simulink model "BCfirsttestwithLPfilter_Simulation"  (Simulink 6.4)
settings: Solver=FixedStepDiscrete  StartTime=0.0  StopTime=1  FixedStep=1/300  RelTol=1e-3
libraries: dspsigops x50
settings Model: Creator=Casparus  LastModifiedBy=lubink
settings OptimizationCC: InlineParams=on  InlineInvariantSignals=on  EnforceIntegerDowncast=off  ZeroExternalMemoryAtStartup=off  ZeroInternalMemoryAtStartup=off  InitFltsAndDblsToZero=off  EfficientFloat2IntCast=on  OptimizeModelRefInitCode=on  LifeSpan=1
settings DebuggingCC: SignalInfNanChecking=error  ReadBeforeWriteMsg=EnableAllAsError  WriteAfterWriteMsg=EnableAllAsError  WriteAfterReadMsg=EnableAllAsError  AlgebraicLoopMsg=error  ArtificialAlgebraicLoopMsg=error  CheckExecutionContextPreStartOutputMsg=on  CheckExecutionContextRuntimeOutputMsg=on  SignalResolutionControl=UseLocalSettings  BlockPriorityViolationMsg=error  SolverPrmCheckMsg=error  InheritedTsInSrcMsg=error  DiscreteInheritContinuousMsg=error  MultiTaskDSMMsg=error  MultiTaskCondExecSysMsg=error  SigSpecEnsureSampleTimeMsg=error  CheckMatrixSingularityMsg=error  ParameterUnderflowMsg=error  ParameterPrecisionLossMsg=error  UnderSpecifiedDataTypeMsg=error  UnnecessaryDatatypeConvMsg=warning  VectorMatrixConversionMsg=error  FcnCallInpInsideContextMsg=Enable All  SignalLabelMismatchMsg=error  UnconnectedInputMsg=error  UnconnectedOutputMsg=error  UnconnectedLineMsg=error  SFcnCompatibilityMsg=error  BusObjectLabelMismatch=error  RootOutportRequireBusObject=error  AssertControl=DisableAll  ModelReferenceIOMsg=error  ModelReferenceIOMismatchMessage=error  ModelReferenceCSMismatchMessage=warning  UnknownTsInhSupMsg=error  ModelReferenceDataLoggingMessage=error
settings HardwareCC: ProdBitPerInt=16  ProdEndianess=LittleEndian  ProdWordSize=16  ProdHWDeviceType=16-bit Generic  TargetHWDeviceType=32-bit Generic
settings RTWCC: SystemTargetFile=dspic.tlc  TemplateMakefile=dspic_pic30_gcc.tmf  PostCodeGenCommand=dsPIC_Compile()  Description=Embedded Target for Microchip dsPIC (real-time)  ProcessScript=dspic_make_rtw_hook
settings CodeAppCC: ForceParamTrailComments=on  IgnoreCustomStorageClasses=off  MangleLength=4  ReqsInCode=on
settings STFCustomTargetCC: TargetFcnLib=ansi_tfl_tmw.mat  GenFloatMathFcnCalls=ANSI_C  ModelReferenceCompliant=off  IncludeMdlTerminateFcn=off  CombineOutputUpdateFcns=on  SuppressErrorStatus=on  ERTCustomFileBanners=on  SupportContinuousTime=off  SupportNonInlinedSFcns=off  SystemTargetFile=dspic.tlc
settings ERTTargetCC: TargetFcnLib=ansi_tfl_tmw.mat  GenFloatMathFcnCalls=ANSI_C  ModelReferenceCompliant=off  CompOptLevelCompliant=off  IncludeMdlTerminateFcn=off  SuppressErrorStatus=on  ModelStepFunctionPrototypeControlCompliant=off  ExtModeMexFile=ext_serial_win32_comm  InlinedParameterPlacement=NonHierarchical  ERTSrcFileBannerTemplate=dsPIC_code_template.cgt  ERTHdrFileBannerTemplate=dsPIC_code_template.cgt  ERTDataSrcFileTemplate=dsPIC_code_template.cgt  ERTDataHdrFileTemplate=dsPIC_code_template.cgt  ERTCustomFileTemplate=dsPIC_main.tlc
settings CustomProperty: DataType=string  Value=C:\PROGRA~1\MATLAB\R2007b\bin\win32\gmake

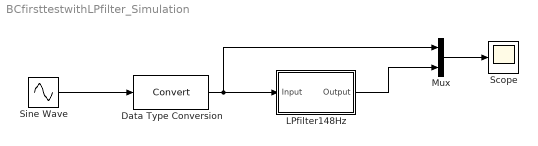
== system BCfirsttestwithLPfilter_Simulation ==
  Data Type Conversion : DataTypeConversion  OutDataTypeMode=uint8  SaturateOnIntegerOverflow=on
  LPfilter148Hz : Subsystem  Tag=FilterWizardSubSystem
      settings: ErrorFcn=dspFilterRealizedInBasicElemsAlgLoopErrFcnCallback
  Mux : Mux  Inputs=2
  Scope : Scope
  Sine Wave : Sin  Amplitude=50  Bias=100  Frequency=30*2*pi  SampleTime=1/300
  wires:
  Sine Wave/1 -> Data Type Conversion/1
  Data Type Conversion/1 -> LPfilter148Hz/1(Input), Mux/1
  LPfilter148Hz/1(Output) -> Mux/2
  Mux/1 -> Scope/1

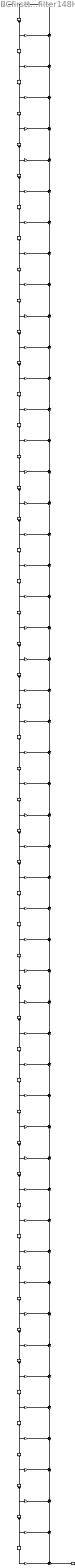
== system BCfirsttestwithLPfilter_Simulation/LPfilter148Hz ==
  Input : Inport
  BodyDelay{2..51} (50 alike) : dspsigops/Delay  Orientation=down  dly_unit=Samples  delay=1  ic_detail=off  dif_ic_for_ch=off  dif_ic_for_dly=off  ic=0  reset_popup=None
  BodyLSum{2..50} (49 alike) : Sum  Orientation=down  Inputs=++|  OutScaling=1  RndMeth=Nearest  SaturateOnIntegerOverflow=on
  BodyLSum51 : Sum  Inputs=++|  OutScaling=1  RndMeth=Nearest  SaturateOnIntegerOverflow=on
  b(1) : Gain  Gain=0.014552788094050004  ParameterDataTypeMode=Specify via dialog  ParameterDataType=float('double')  OutScaling=1  RndMeth=Nearest  SaturateOnIntegerOverflow=on
  b(10) : Gain  Gain=0.009640191238745691  ParameterDataTypeMode=Specify via dialog  ParameterDataType=float('double')  OutScaling=1  RndMeth=Nearest  SaturateOnIntegerOverflow=on
  b(11) : Gain  Gain=-0.0085605708557222188  ParameterDataTypeMode=Specify via dialog  ParameterDataType=float('double')  OutScaling=1  RndMeth=Nearest  SaturateOnIntegerOverflow=on
  b(12) : Gain  Gain=0.0063507327962420345  ParameterDataTypeMode=Specify via dialog  ParameterDataType=float('double')  OutScaling=1  RndMeth=Nearest  SaturateOnIntegerOverflow=on
  b(13) : Gain  Gain=-0.0029026251186017836  ParameterDataTypeMode=Specify via dialog  ParameterDataType=float('double')  OutScaling=1  RndMeth=Nearest  SaturateOnIntegerOverflow=on
  b(14) : Gain  Gain=-0.0018214634792136299  ParameterDataTypeMode=Specify via dialog  ParameterDataType=float('double')  OutScaling=1  RndMeth=Nearest  SaturateOnIntegerOverflow=on
  b(15) : Gain  Gain=0.0077807436385992461  ParameterDataTypeMode=Specify via dialog  ParameterDataType=float('double')  OutScaling=1  RndMeth=Nearest  SaturateOnIntegerOverflow=on
  b(16) : Gain  Gain=-0.014854401199296334  ParameterDataTypeMode=Specify via dialog  ParameterDataType=float('double')  OutScaling=1  RndMeth=Nearest  SaturateOnIntegerOverflow=on
  b(17) : Gain  Gain=0.022857994519878629  ParameterDataTypeMode=Specify via dialog  ParameterDataType=float('double')  OutScaling=1  RndMeth=Nearest  SaturateOnIntegerOverflow=on
  b(18) : Gain  Gain=-0.031505854072013589  ParameterDataTypeMode=Specify via dialog  ParameterDataType=float('double')  OutScaling=1  RndMeth=Nearest  SaturateOnIntegerOverflow=on
  b(19) : Gain  Gain=0.040407776537517141  ParameterDataTypeMode=Specify via dialog  ParameterDataType=float('double')  OutScaling=1  RndMeth=Nearest  SaturateOnIntegerOverflow=on
  b(2) : Gain  Gain=0.001488942337451464  ParameterDataTypeMode=Specify via dialog  ParameterDataType=float('double')  OutScaling=1  RndMeth=Nearest  SaturateOnIntegerOverflow=on
  b(20) : Gain  Gain=-0.049274632193230417  ParameterDataTypeMode=Specify via dialog  ParameterDataType=float('double')  OutScaling=1  RndMeth=Nearest  SaturateOnIntegerOverflow=on
  b(21) : Gain  Gain=0.057661319766925831  ParameterDataTypeMode=Specify via dialog  ParameterDataType=float('double')  OutScaling=1  RndMeth=Nearest  SaturateOnIntegerOverflow=on
  b(22) : Gain  Gain=-0.065171220365631818  ParameterDataTypeMode=Specify via dialog  ParameterDataType=float('double')  OutScaling=1  RndMeth=Nearest  SaturateOnIntegerOverflow=on
  b(23) : Gain  Gain=0.0714398868910541  ParameterDataTypeMode=Specify via dialog  ParameterDataType=float('double')  OutScaling=1  RndMeth=Nearest  SaturateOnIntegerOverflow=on
  b(24) : Gain  Gain=-0.076157677489708669  ParameterDataTypeMode=Specify via dialog  ParameterDataType=float('double')  OutScaling=1  RndMeth=Nearest  SaturateOnIntegerOverflow=on
  b(25) : Gain  Gain=0.079087854814890529  ParameterDataTypeMode=Specify via dialog  ParameterDataType=float('double')  OutScaling=1  RndMeth=Nearest  SaturateOnIntegerOverflow=on
  b(26) : Gain  Gain=0.91991847348550915  ParameterDataTypeMode=Specify via dialog  ParameterDataType=float('double')  OutScaling=1  RndMeth=Nearest  SaturateOnIntegerOverflow=on
  b(27) : Gain  Gain=0.079087854814890529  ParameterDataTypeMode=Specify via dialog  ParameterDataType=float('double')  OutScaling=1  RndMeth=Nearest  SaturateOnIntegerOverflow=on
  b(28) : Gain  Gain=-0.076157677489708669  ParameterDataTypeMode=Specify via dialog  ParameterDataType=float('double')  OutScaling=1  RndMeth=Nearest  SaturateOnIntegerOverflow=on
  b(29) : Gain  Gain=0.0714398868910541  ParameterDataTypeMode=Specify via dialog  ParameterDataType=float('double')  OutScaling=1  RndMeth=Nearest  SaturateOnIntegerOverflow=on
  b(3) : Gain  Gain=-0.0022367192816874449  ParameterDataTypeMode=Specify via dialog  ParameterDataType=float('double')  OutScaling=1  RndMeth=Nearest  SaturateOnIntegerOverflow=on
  b(30) : Gain  Gain=-0.065171220365631818  ParameterDataTypeMode=Specify via dialog  ParameterDataType=float('double')  OutScaling=1  RndMeth=Nearest  SaturateOnIntegerOverflow=on
  b(31) : Gain  Gain=0.057661319766925831  ParameterDataTypeMode=Specify via dialog  ParameterDataType=float('double')  OutScaling=1  RndMeth=Nearest  SaturateOnIntegerOverflow=on
  b(32) : Gain  Gain=-0.049274632193230417  ParameterDataTypeMode=Specify via dialog  ParameterDataType=float('double')  OutScaling=1  RndMeth=Nearest  SaturateOnIntegerOverflow=on
  b(33) : Gain  Gain=0.040407776537517141  ParameterDataTypeMode=Specify via dialog  ParameterDataType=float('double')  OutScaling=1  RndMeth=Nearest  SaturateOnIntegerOverflow=on
  b(34) : Gain  Gain=-0.031505854072013589  ParameterDataTypeMode=Specify via dialog  ParameterDataType=float('double')  OutScaling=1  RndMeth=Nearest  SaturateOnIntegerOverflow=on
  b(35) : Gain  Gain=0.022857994519878629  ParameterDataTypeMode=Specify via dialog  ParameterDataType=float('double')  OutScaling=1  RndMeth=Nearest  SaturateOnIntegerOverflow=on
  b(36) : Gain  Gain=-0.014854401199296334  ParameterDataTypeMode=Specify via dialog  ParameterDataType=float('double')  OutScaling=1  RndMeth=Nearest  SaturateOnIntegerOverflow=on
  b(37) : Gain  Gain=0.0077807436385992461  ParameterDataTypeMode=Specify via dialog  ParameterDataType=float('double')  OutScaling=1  RndMeth=Nearest  SaturateOnIntegerOverflow=on
  b(38) : Gain  Gain=-0.0018214634792136299  ParameterDataTypeMode=Specify via dialog  ParameterDataType=float('double')  OutScaling=1  RndMeth=Nearest  SaturateOnIntegerOverflow=on
  b(39) : Gain  Gain=-0.0029026251186017836  ParameterDataTypeMode=Specify via dialog  ParameterDataType=float('double')  OutScaling=1  RndMeth=Nearest  SaturateOnIntegerOverflow=on
  b(4) : Gain  Gain=0.0033999777744855996  ParameterDataTypeMode=Specify via dialog  ParameterDataType=float('double')  OutScaling=1  RndMeth=Nearest  SaturateOnIntegerOverflow=on
  b(40) : Gain  Gain=0.0063507327962420345  ParameterDataTypeMode=Specify via dialog  ParameterDataType=float('double')  OutScaling=1  RndMeth=Nearest  SaturateOnIntegerOverflow=on
  b(41) : Gain  Gain=-0.0085605708557222188  ParameterDataTypeMode=Specify via dialog  ParameterDataType=float('double')  OutScaling=1  RndMeth=Nearest  SaturateOnIntegerOverflow=on
  b(42) : Gain  Gain=0.009640191238745691  ParameterDataTypeMode=Specify via dialog  ParameterDataType=float('double')  OutScaling=1  RndMeth=Nearest  SaturateOnIntegerOverflow=on
  b(43) : Gain  Gain=-0.0097539264573168211  ParameterDataTypeMode=Specify via dialog  ParameterDataType=float('double')  OutScaling=1  RndMeth=Nearest  SaturateOnIntegerOverflow=on
  b(44) : Gain  Gain=0.0091052834705578258  ParameterDataTypeMode=Specify via dialog  ParameterDataType=float('double')  OutScaling=1  RndMeth=Nearest  SaturateOnIntegerOverflow=on
  b(45) : Gain  Gain=-0.0079195888626813621  ParameterDataTypeMode=Specify via dialog  ParameterDataType=float('double')  OutScaling=1  RndMeth=Nearest  SaturateOnIntegerOverflow=on
  b(46) : Gain  Gain=0.0064281050997838478  ParameterDataTypeMode=Specify via dialog  ParameterDataType=float('double')  OutScaling=1  RndMeth=Nearest  SaturateOnIntegerOverflow=on
  b(47) : Gain  Gain=-0.0048540570262981418  ParameterDataTypeMode=Specify via dialog  ParameterDataType=float('double')  OutScaling=1  RndMeth=Nearest  SaturateOnIntegerOverflow=on
  b(48) : Gain  Gain=0.0033999777744855996  ParameterDataTypeMode=Specify via dialog  ParameterDataType=float('double')  OutScaling=1  RndMeth=Nearest  SaturateOnIntegerOverflow=on
  b(49) : Gain  Gain=-0.0022367192816874449  ParameterDataTypeMode=Specify via dialog  ParameterDataType=float('double')  OutScaling=1  RndMeth=Nearest  SaturateOnIntegerOverflow=on
  b(5) : Gain  Gain=-0.0048540570262981418  ParameterDataTypeMode=Specify via dialog  ParameterDataType=float('double')  OutScaling=1  RndMeth=Nearest  SaturateOnIntegerOverflow=on
  b(50) : Gain  Gain=0.001488942337451464  ParameterDataTypeMode=Specify via dialog  ParameterDataType=float('double')  OutScaling=1  RndMeth=Nearest  SaturateOnIntegerOverflow=on
  b(51) : Gain  Gain=0.014552788094050004  ParameterDataTypeMode=Specify via dialog  ParameterDataType=float('double')  OutScaling=1  RndMeth=Nearest  SaturateOnIntegerOverflow=on
  b(6) : Gain  Gain=0.0064281050997838478  ParameterDataTypeMode=Specify via dialog  ParameterDataType=float('double')  OutScaling=1  RndMeth=Nearest  SaturateOnIntegerOverflow=on
  b(7) : Gain  Gain=-0.0079195888626813621  ParameterDataTypeMode=Specify via dialog  ParameterDataType=float('double')  OutScaling=1  RndMeth=Nearest  SaturateOnIntegerOverflow=on
  b(8) : Gain  Gain=0.0091052834705578258  ParameterDataTypeMode=Specify via dialog  ParameterDataType=float('double')  OutScaling=1  RndMeth=Nearest  SaturateOnIntegerOverflow=on
  b(9) : Gain  Gain=-0.0097539264573168211  ParameterDataTypeMode=Specify via dialog  ParameterDataType=float('double')  OutScaling=1  RndMeth=Nearest  SaturateOnIntegerOverflow=on
  Output : Outport
  wires:
  BodyLSum51/1 -> Output/1
  b(51)/1 -> BodyLSum51/2
  BodyDelay51/1 -> b(51)/1
  BodyLSum50/1 -> BodyLSum51/1
  b(50)/1 -> BodyLSum50/1
  BodyDelay50/1 -> BodyDelay51/1, b(50)/1
  BodyLSum49/1 -> BodyLSum50/2
  b(49)/1 -> BodyLSum49/1
  BodyDelay49/1 -> BodyDelay50/1, b(49)/1
  BodyLSum48/1 -> BodyLSum49/2
  b(48)/1 -> BodyLSum48/1
  BodyDelay48/1 -> BodyDelay49/1, b(48)/1
  BodyLSum47/1 -> BodyLSum48/2
  b(47)/1 -> BodyLSum47/1
  BodyDelay47/1 -> BodyDelay48/1, b(47)/1
  BodyLSum46/1 -> BodyLSum47/2
  b(46)/1 -> BodyLSum46/1
  BodyDelay46/1 -> BodyDelay47/1, b(46)/1
  BodyLSum45/1 -> BodyLSum46/2
  b(45)/1 -> BodyLSum45/1
  BodyDelay45/1 -> BodyDelay46/1, b(45)/1
  BodyLSum44/1 -> BodyLSum45/2
  b(44)/1 -> BodyLSum44/1
  BodyDelay44/1 -> BodyDelay45/1, b(44)/1
  BodyLSum43/1 -> BodyLSum44/2
  b(43)/1 -> BodyLSum43/1
  BodyDelay43/1 -> BodyDelay44/1, b(43)/1
  BodyLSum42/1 -> BodyLSum43/2
  b(42)/1 -> BodyLSum42/1
  BodyDelay42/1 -> BodyDelay43/1, b(42)/1
  BodyLSum41/1 -> BodyLSum42/2
  b(41)/1 -> BodyLSum41/1
  BodyDelay41/1 -> BodyDelay42/1, b(41)/1
  BodyLSum40/1 -> BodyLSum41/2
  b(40)/1 -> BodyLSum40/1
  BodyDelay40/1 -> BodyDelay41/1, b(40)/1
  BodyLSum39/1 -> BodyLSum40/2
  b(39)/1 -> BodyLSum39/1
  BodyDelay39/1 -> BodyDelay40/1, b(39)/1
  BodyLSum38/1 -> BodyLSum39/2
  b(38)/1 -> BodyLSum38/1
  BodyDelay38/1 -> BodyDelay39/1, b(38)/1
  BodyLSum37/1 -> BodyLSum38/2
  b(37)/1 -> BodyLSum37/1
  BodyDelay37/1 -> BodyDelay38/1, b(37)/1
  BodyLSum36/1 -> BodyLSum37/2
  b(36)/1 -> BodyLSum36/1
  BodyDelay36/1 -> BodyDelay37/1, b(36)/1
  BodyLSum35/1 -> BodyLSum36/2
  b(35)/1 -> BodyLSum35/1
  BodyDelay35/1 -> BodyDelay36/1, b(35)/1
  BodyLSum34/1 -> BodyLSum35/2
  b(34)/1 -> BodyLSum34/1
  BodyDelay34/1 -> BodyDelay35/1, b(34)/1
  BodyLSum33/1 -> BodyLSum34/2
  b(33)/1 -> BodyLSum33/1
  BodyDelay33/1 -> BodyDelay34/1, b(33)/1
  BodyLSum32/1 -> BodyLSum33/2
  b(32)/1 -> BodyLSum32/1
  BodyDelay32/1 -> BodyDelay33/1, b(32)/1
  BodyLSum31/1 -> BodyLSum32/2
  b(31)/1 -> BodyLSum31/1
  BodyDelay31/1 -> BodyDelay32/1, b(31)/1
  BodyLSum30/1 -> BodyLSum31/2
  b(30)/1 -> BodyLSum30/1
  BodyDelay30/1 -> BodyDelay31/1, b(30)/1
  BodyLSum29/1 -> BodyLSum30/2
  b(29)/1 -> BodyLSum29/1
  BodyDelay29/1 -> BodyDelay30/1, b(29)/1
  BodyLSum28/1 -> BodyLSum29/2
  b(28)/1 -> BodyLSum28/1
  BodyDelay28/1 -> BodyDelay29/1, b(28)/1
  BodyLSum27/1 -> BodyLSum28/2
  b(27)/1 -> BodyLSum27/1
  BodyDelay27/1 -> BodyDelay28/1, b(27)/1
  BodyLSum26/1 -> BodyLSum27/2
  b(26)/1 -> BodyLSum26/1
  BodyDelay26/1 -> BodyDelay27/1, b(26)/1
  BodyLSum25/1 -> BodyLSum26/2
  b(25)/1 -> BodyLSum25/1
  BodyDelay25/1 -> BodyDelay26/1, b(25)/1
  BodyLSum24/1 -> BodyLSum25/2
  b(24)/1 -> BodyLSum24/1
  BodyDelay24/1 -> BodyDelay25/1, b(24)/1
  BodyLSum23/1 -> BodyLSum24/2
  b(23)/1 -> BodyLSum23/1
  BodyDelay23/1 -> BodyDelay24/1, b(23)/1
  BodyLSum22/1 -> BodyLSum23/2
  b(22)/1 -> BodyLSum22/1
  BodyDelay22/1 -> BodyDelay23/1, b(22)/1
  BodyLSum21/1 -> BodyLSum22/2
  b(21)/1 -> BodyLSum21/1
  BodyDelay21/1 -> BodyDelay22/1, b(21)/1
  BodyLSum20/1 -> BodyLSum21/2
  b(20)/1 -> BodyLSum20/1
  BodyDelay20/1 -> BodyDelay21/1, b(20)/1
  BodyLSum19/1 -> BodyLSum20/2
  b(19)/1 -> BodyLSum19/1
  BodyDelay19/1 -> BodyDelay20/1, b(19)/1
  BodyLSum18/1 -> BodyLSum19/2
  b(18)/1 -> BodyLSum18/1
  BodyDelay18/1 -> BodyDelay19/1, b(18)/1
  BodyLSum17/1 -> BodyLSum18/2
  b(17)/1 -> BodyLSum17/1
  BodyDelay17/1 -> BodyDelay18/1, b(17)/1
  BodyLSum16/1 -> BodyLSum17/2
  b(16)/1 -> BodyLSum16/1
  BodyDelay16/1 -> BodyDelay17/1, b(16)/1
  BodyLSum15/1 -> BodyLSum16/2
  b(15)/1 -> BodyLSum15/1
  BodyDelay15/1 -> BodyDelay16/1, b(15)/1
  BodyLSum14/1 -> BodyLSum15/2
  b(14)/1 -> BodyLSum14/1
  BodyDelay14/1 -> BodyDelay15/1, b(14)/1
  BodyLSum13/1 -> BodyLSum14/2
  b(13)/1 -> BodyLSum13/1
  BodyDelay13/1 -> BodyDelay14/1, b(13)/1
  BodyLSum12/1 -> BodyLSum13/2
  b(12)/1 -> BodyLSum12/1
  BodyDelay12/1 -> BodyDelay13/1, b(12)/1
  BodyLSum11/1 -> BodyLSum12/2
  b(11)/1 -> BodyLSum11/1
  BodyDelay11/1 -> BodyDelay12/1, b(11)/1
  BodyLSum10/1 -> BodyLSum11/2
  b(10)/1 -> BodyLSum10/1
  BodyDelay10/1 -> BodyDelay11/1, b(10)/1
  BodyLSum9/1 -> BodyLSum10/2
  b(9)/1 -> BodyLSum9/1
  BodyDelay9/1 -> BodyDelay10/1, b(9)/1
  BodyLSum8/1 -> BodyLSum9/2
  b(8)/1 -> BodyLSum8/1
  BodyDelay8/1 -> BodyDelay9/1, b(8)/1
  BodyLSum7/1 -> BodyLSum8/2
  b(7)/1 -> BodyLSum7/1
  BodyDelay7/1 -> BodyDelay8/1, b(7)/1
  BodyLSum6/1 -> BodyLSum7/2
  b(6)/1 -> BodyLSum6/1
  BodyDelay6/1 -> BodyDelay7/1, b(6)/1
  BodyLSum5/1 -> BodyLSum6/2
  b(5)/1 -> BodyLSum5/1
  BodyDelay5/1 -> BodyDelay6/1, b(5)/1
  BodyLSum4/1 -> BodyLSum5/2
  b(4)/1 -> BodyLSum4/1
  BodyDelay4/1 -> BodyDelay5/1, b(4)/1
  BodyLSum3/1 -> BodyLSum4/2
  b(3)/1 -> BodyLSum3/1
  BodyDelay3/1 -> BodyDelay4/1, b(3)/1
  BodyLSum2/1 -> BodyLSum3/2
  b(2)/1 -> BodyLSum2/1
  BodyDelay2/1 -> BodyDelay3/1, b(2)/1
  b(1)/1 -> BodyLSum2/2
  Input/1 -> BodyDelay2/1, b(1)/1
